simulink model "ProjetACC_Master_senario2"  (R2026a)
settings: Solver=VariableStepAuto  StopTime=120
values from neighbouring files (symbols this model uses):
  acc_frein = -2    [parametres_acc.m]
  acc_max = 1.5    [parametres_acc.m]
  acc_min = -4    [parametres_acc.m]
  acc_reprise = 1    [parametres_acc.m]
  dist_arret = 6    [parametres_acc.m]
  duree_frein = 5    [parametres_acc.m]
  duree_reprise = 10    [parametres_acc.m]
  ecart_temps = 1.8    [parametres_acc.m]
  Kp_d = 0.2    [parametres_acc.m]
  Kp_v = 0.5    [parametres_acc.m]
  Kv = 0.8    [parametres_acc.m]
  pos0_suiv = 0    [parametres_acc.m]
  pos0_tete = 70    [parametres_acc.m]
  t_cutin = 90    [parametres_acc.m]
  t_frein = 30    [parametres_acc.m]
  t_reprise = 60    [parametres_acc.m]
  tau_veh = 0.8    [parametres_acc.m]
  vit0_suiv = 15    [parametres_acc.m]
  vit0_tete = 22    [parametres_acc.m]
  vit_consigne = 27    [parametres_acc.m]
settings Model: Creator=AYOUB MK  LastModifiedBy=AYOUB MK

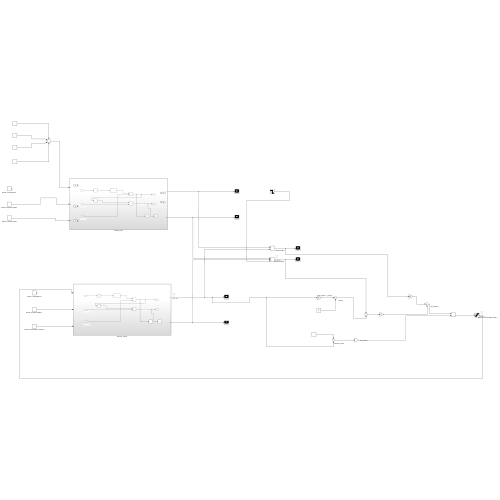
[thumbnail: Simulink's stored preview of the top-level diagram]
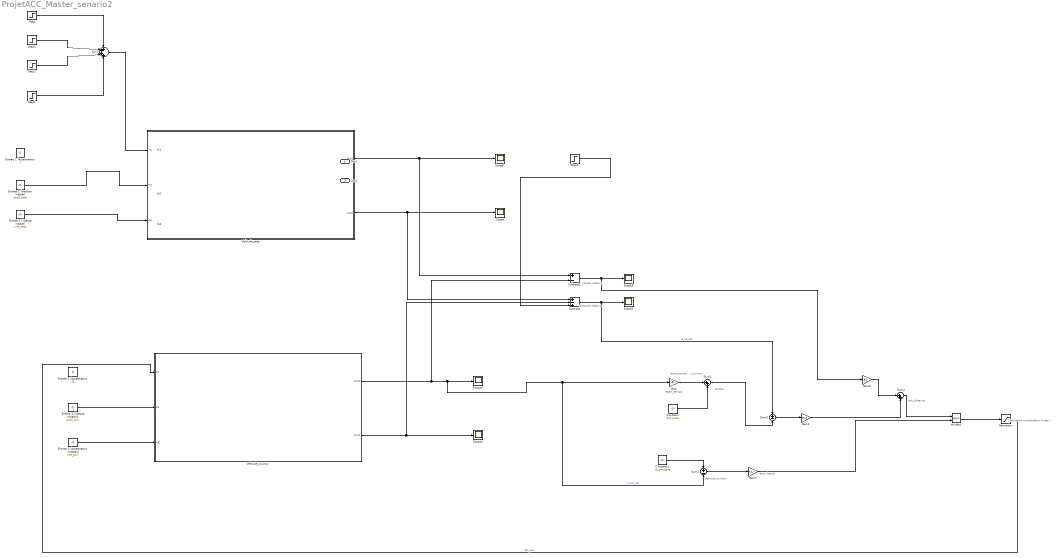
== system ProjetACC_Master_senario2 ==
  note: Saturation (accélération finale )
  note: acc_distance
  note: acc_vitesse
  note: Vehicule_suiveur
  note: ecart_temps · v_suiveur
  note: D-safe
  note: distance relative
  note: vitesse relative
  In1 : Inport
  In2 : Inport  Port=2
  In3 : Inport  Port=3
  Constant : Constant  Value=dist_arret
  Constant1 : Constant  Value=vit_consigne
  Entrée 1 (accélération) : Constant  Value=0
  Entrée 1 (accélération)1 : Constant  Value=0
  Entrée 2 (position initiale) : Constant  Value=pos0_tete
  Entrée 3 (acceleration  initiale)2 : Constant  Value=vit0_suiv
  Entrée 3 (vitesse initiale) : Constant  Value=vit0_tete
  Entrée 3 (vitesse initiale)1 : Constant  Value=pos0_suiv
  Gain : Gain  Gain=ecart_temps
  Gain1 : Gain  Gain=Kp_v
  Gain2 : Gain  Gain=Kp_d
  Gain3 : Gain  Gain=Kv
  MinMax : MinMax  Inputs=2
  Saturation : Saturate  UpperLimit=acc_max  LowerLimit=acc_min
  Scope{,1..5} (6 alike) : Scope
      Scope settings: ActiveDisplayYMinimum=-1  ActiveDisplayYMaximum=1
      Scope1 settings: ActiveDisplayYMinimum=-1  ActiveDisplayYMaximum=1
      Scope2 settings: ActiveDisplayYMinimum=-535.1483282234982  ActiveDisplayYMaximum=2916.6764436425569  DataLoggingVariableName=ScopeData4
      Scope3 settings: ActiveDisplayYMinimum=-1  ActiveDisplayYMaximum=1  DataLoggingVariableName=ScopeData5
      Scope4 settings: ActiveDisplayYMinimum=-116.30350931859374  ActiveDisplayYMaximum=957.48600460530156  DataLoggingVariableName=ScopeData6
      Scope5 settings: ActiveDisplayYMinimum=-1  ActiveDisplayYMaximum=1  DataLoggingVariableName=ScopeData7
  Step : Step  Time=t_frein  FinalValue=acc_frein  SampleTime=0
  Step1 : Step  Time=t_reprise + duree_reprise  FinalValue=-acc_reprise  SampleTime=0
  Step2 : Step  Time=t_reprise  FinalValue=acc_reprise  SampleTime=0
  Step3 : Step  Time=t_frein + duree_frein  FinalValue=-acc_frein  SampleTime=0
  Step4 : Step  Time=t_cutin  FinalValue=delta_cutin  SampleTime=0
  Subtract : Sum  Inputs=+-+
  Subtract1 : Sum  Inputs=+-
  Sum : Sum  Inputs=++++
  Sum1 : Sum  Inputs=|++
  Sum2 : Sum  Inputs=+-
  Sum3 : Sum  Inputs=+-
  Sum4 : Sum  Inputs=|++
  Vehicule_suiveur : Subsystem
  Vehicule_tete : Subsystem
  Out1 : Outport
  Out2 : Outport  Port=2
  wires:
  Entrée 2 (position initiale)/1 -> Vehicule_tete/2(In2)
  Entrée 3 (vitesse initiale)/1 -> Vehicule_tete/3(In3)
  Step1/1 -> Sum/4
  Step2/1 -> Sum/3
  Step3/1 -> Sum/2
  Step/1 -> Sum/1
  Sum/1 -> Vehicule_tete/1(In1)
  Vehicule_tete/2(Out2) -> Scope/1, Subtract/1
  Vehicule_tete/1(Out1) -> Scope1/1, Subtract1/1
  Entrée 3 (acceleration  initiale)2/1 -> Vehicule_suiveur/3(In3)
  Entrée 3 (vitesse initiale)1/1 -> Vehicule_suiveur/2(In2)
  Vehicule_suiveur/1(Out1) -> Subtract1/2, Sum2/2, Gain/1, Scope3/1  "v_suiv_out"
  Vehicule_suiveur/2(Out2) -> Subtract/2, Scope2/1
  Subtract/1 -> Scope4/1, Sum3/1  "d_rel_out"
  Subtract1/1 -> Scope5/1, Gain3/1
  Gain/1 -> Sum1/1
  Constant/1 -> Sum1/2
  Constant1/1 -> Sum2/1
  Sum2/1 -> Gain1/1
  Sum1/1 -> Sum3/2
  Sum3/1 -> Gain2/1
  Gain2/1 -> Sum4/2
  Gain3/1 -> Sum4/1
  Sum4/1 -> MinMax/1
  Gain1/1 -> MinMax/2
  MinMax/1 -> Saturation/1
  Saturation/1 -> Vehicule_suiveur/1(In1)  "acc_suiv"
  Step4/1 -> Subtract/3

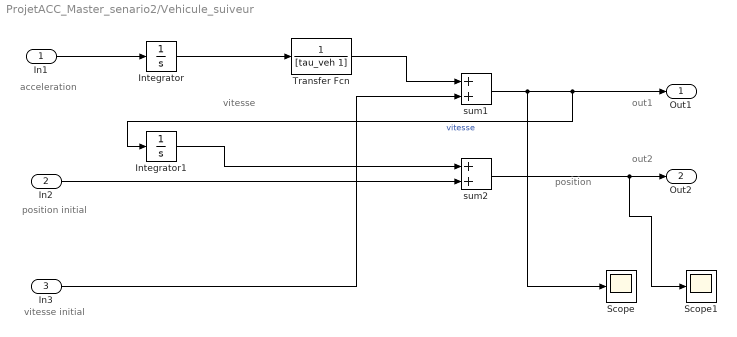
== system ProjetACC_Master_senario2/Vehicule_suiveur ==
  note: vitesse
  note: position
  note: position initial
  note: out2
  note: out1
  note: vitesse initial
  note: acceleration
  In1 : Inport
  In2 : Inport  Port=2
  In3 : Inport  Port=3
  Integrator : Integrator
  Integrator1 : Integrator
  Scope : Scope
      settings: ActiveDisplayYMinimum=5  ActiveDisplayYMaximum=25  DataLoggingVariableName=ScopeData2
  Scope1 : Scope
      settings: ActiveDisplayYMinimum=-1  ActiveDisplayYMaximum=1  DataLoggingVariableName=ScopeData3
  Transfer Fcn : TransferFcn  Denominator=[tau_veh 1]
  sum1 : Sum
  sum2 : Sum
  Out1 : Outport
  Out2 : Outport  Port=2
  wires:
  Integrator1/1 -> sum2/1
  Integrator/1 -> Transfer Fcn/1
  sum1/1 -> Scope/1, Integrator1/1, Out1/1  "vitesse"
  In3/1 -> sum1/2
  In2/1 -> sum2/2
  In1/1 -> Integrator/1
  Transfer Fcn/1 -> sum1/1
  sum2/1 -> Scope1/1, Out2/1

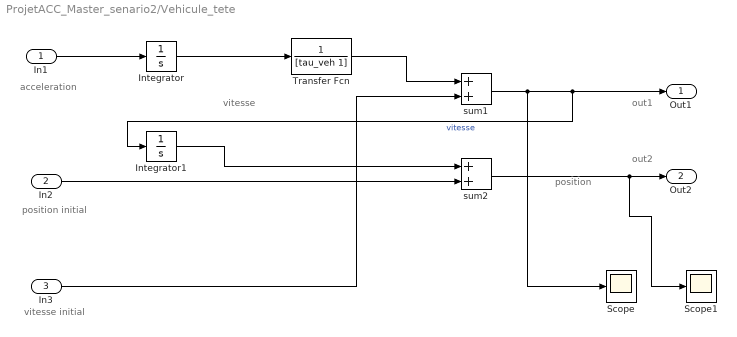
== system ProjetACC_Master_senario2/Vehicule_tete ==
  note: vitesse
  note: position
  note: position initial
  note: out2
  note: out1
  note: vitesse initial
  note: acceleration
  In1 : Inport
  In2 : Inport  Port=2
  In3 : Inport  Port=3
  Integrator : Integrator
  Integrator1 : Integrator
  Scope : Scope
      settings: ActiveDisplayYMinimum=-1  ActiveDisplayYMaximum=1  DataLoggingVariableName=ScopeData2
  Scope1 : Scope
      settings: ActiveDisplayYMinimum=-1  ActiveDisplayYMaximum=1  DataLoggingVariableName=ScopeData3
  Transfer Fcn : TransferFcn  Denominator=[tau_veh 1]
  sum1 : Sum
  sum2 : Sum
  Out1 : Outport
  Out2 : Outport  Port=2
  wires:
  Integrator1/1 -> sum2/1
  Integrator/1 -> Transfer Fcn/1
  sum1/1 -> Scope/1, Integrator1/1, Out1/1  "vitesse"
  In3/1 -> sum1/2
  In2/1 -> sum2/2
  In1/1 -> Integrator/1
  Transfer Fcn/1 -> sum1/1
  sum2/1 -> Scope1/1, Out2/1
